simulink model "IEEE_BUS_68_AGC"  (R2025a)
settings: Solver=ode23tb  StartTime=0.0  StopTime=150  FixedStep=Ts  MaxStep=0.0001  RelTol=1e-3
PreLoadFcn:
  | PSSMODEL=1;
  | LPSS=0;
  | WAPSS=0;
  | WAPSS2=0;
  | Ts=50e-5;
InitFcn:
  | PSSMODEL=1;
  | LPSS=0;
  | WAPSS=0;
  | WAPSS2=0;
  | Ts=50e-5;
  | 
  | % Required data to 68 Bus benchmark
  | % clear
  | % clc
  | % Definition for the columns
  | % system base =100 MVA
  | 
  | %% Line data Format (line)
  | % All values are given on the same system base MVA
  | % 1: From bus
  | % 2: To bus
  | % 3: Resistance (pu)
  | % 4: Reactance  (pu)
  | % 5: Charge     (pu)
  | % 6: Transformer Tap Amplitute
  | % 7: base MVA
  | % 8: Nomonal Voltage (KV)
  | 
  | %1   2    3        4       5       6        7      8
  | line=[...
  | 1	54	0	     0.0181	  0	      1.025     100    13.8
  | 2	58	0	     0.025	  0	      1.070     100    13.8
  | 3	62	0	     0.02	  0	      1.070     100    13.8
  | 4	19	0.0007	 0.0142	  0	      1.070     100    13.8
  | 5	20	0.0009	 0.018	  0	      1.009     100    13.8
  | 6	22	0	     0.0143	  0	      1.025     100    13.8
  | 7	23	0.0005	 0.0272	  0	      0         100    13.8
  | 8	25	0.0006	 0.0232	  0	      1.025     100    13.8
  | 9	29	0.0008	 0.0156   0	      1.025     100    13.8
  | 10	31	0	     0.026	  0	      1.04      100    13.8
  | 11	32	0	     0.013	  0	      1.04      100    13.8
  | 12	36	0	     0.0075	  0	      1.04      100    13.8
  | 13	17	0	     0.0033	  0	      1.04      100    13.8
  | 14	41	0	     0.0015	  0	      1         100    13.8
  | 15	42	0	     0.0015	  0	      1         100    13.8
  | 16	18	0	     0.003	  0	      1         100    13.8
  | 17	36	0.0005	 0.0045	  0.32	  0         100    138
  | 17	43	0.0005	 0.0276	  0	      0         100    138
  | 18	42	0.004	 0.06	  2.25    0         100    138
  | 18	49	0.0076	 0.1141	  1.16    0	        100    138
  | 18	50	0.0012	 0.0288	  2.06	  0         100    138
  | 20	19	0.0007	 0.0138	  0       1.06	    100    138
  | 19	68	0.0016	 0.0195	  0.304	  0         100    138
  | 21	22	0.0008	 0.014	  0.2565  0	        100    138
  | 21	68	0.0008	 0.0135	  0.2548  0	        100    138
  | 22	23	0.0006	 0.0096	  0.1846  0	        100    138
  | 23	24	0.0022	 0.035	  0.361	  0         100    138
  | 24	68	0.0003	 0.0059	  0.068	  0         100    138
  | 25	26	0.0032	 0.0323	  0.531	  0         100    138
  | 25	54	0.007	 0.0086	  0.146	  0         100    138
  | 26	27	0.0014	 0.0147	  0.2396  0	        100    138
  | 26	28	0.0043	 0.0474	  0.7802  0	        100    138
  | 26	29	0.0057	 0.0625	  1.029	  0         100    138
  | 27	37	0.0013	 0.0173	  0.3216  0	        100    138
  | 27	53	0.032	 0.32	  0.41	  0         100    138
  | ... (+206 lines)
undefined symbols (not defined in the file or in its folder): D1, Delta
libraries: spsPMUPLLBasedPositiveSequenceLib x90, spsRMSLib x73, spsThreePhaseVIMeasurementLib x69, spsLoadFlowBusLib x69, spsThreePhasePISectionLineLib x64, spsThreePhaseParallelRLCLoadLib x35, spsGenericPowerSystemStabilizerLib x32, spsThreePhaseSeriesRLCLoadLib x21, spsThreePhaseTransformerTwoWindingsLib x21, spsSynchronousMachinepuStandardLib x20, spsExcitationSystemLib x16, spsMultiBandPowerSystemStabilizerLib x16
(part 4 of 8)

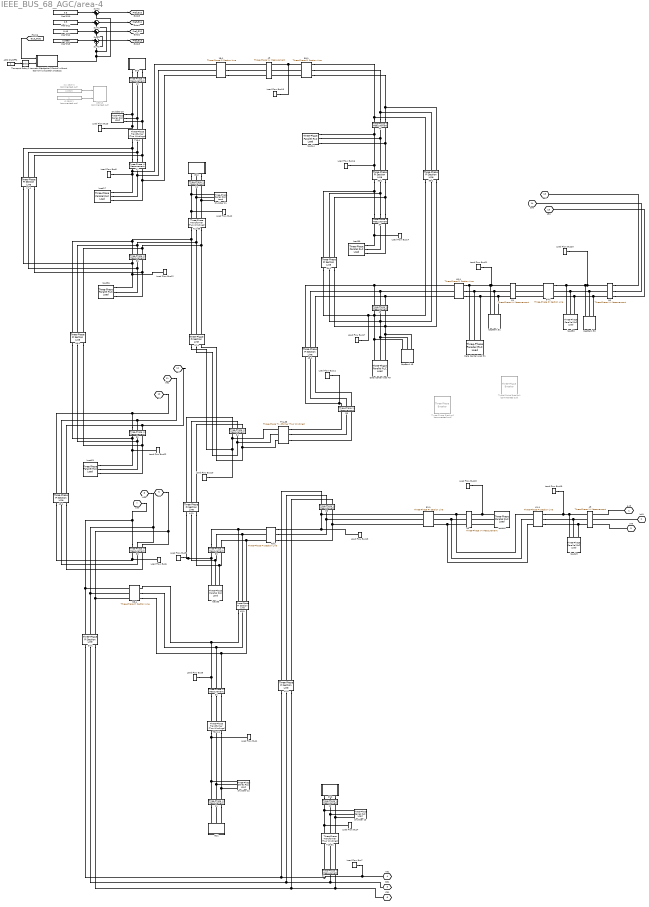
== system IEEE_BUS_68_AGC/area-4 ==
  10 : spsThreePhaseVIMeasurementLib/Three-Phase V-I Measurement  VoltageMeasurement=phase-to-phase  SetLabelV=on  LabelV=Vabc_10  Vpu=off  VpuLL=on  CurrentMeasurement=no  SetLabelI=off  LabelI=Iabc  Ipu=off  Pbase=100e6  Vbase=13.8e3  OutputType=Complex  PhasorSimulation=off  PSBequivalent=0
  11 : spsThreePhaseVIMeasurementLib/Three-Phase V-I Measurement  VoltageMeasurement=phase-to-phase  SetLabelV=on  LabelV=Vabc_11  Vpu=off  VpuLL=on  CurrentMeasurement=no  SetLabelI=off  LabelI=Iabc  Ipu=off  Pbase=100e6  Vbase=13.8e3  OutputType=Complex  PhasorSimulation=off  PSBequivalent=0
  12 : spsThreePhaseVIMeasurementLib/Three-Phase V-I Measurement  VoltageMeasurement=phase-to-phase  SetLabelV=on  LabelV=Vabc_12  Vpu=off  VpuLL=on  CurrentMeasurement=no  SetLabelI=off  LabelI=Iabc  Ipu=off  Pbase=100e6  Vbase=13.8e3  OutputType=Complex  PhasorSimulation=off  PSBequivalent=0
  13 : spsThreePhaseVIMeasurementLib/Three-Phase V-I Measurement  VoltageMeasurement=phase-to-phase  SetLabelV=on  LabelV=Vabc_13  Vpu=off  VpuLL=on  CurrentMeasurement=no  SetLabelI=off  LabelI=Iabc  Ipu=off  Pbase=100e6  Vbase=13.8e3  OutputType=Complex  PhasorSimulation=off  PSBequivalent=0
  17 : spsThreePhaseVIMeasurementLib/Three-Phase V-I Measurement  VoltageMeasurement=phase-to-phase  SetLabelV=on  LabelV=Vabc_17  Vpu=off  VpuLL=on  CurrentMeasurement=no  SetLabelI=off  LabelI=Iabc  Ipu=off  Pbase=100e6  Vbase=Bus(17,2)*1e3  OutputType=Complex  PhasorSimulation=off  PSBequivalent=0
  17-1 : spsThreePhasePISectionLineLib/Three-Phase PI Section Line  LConnTagsString=a|b|c  RConnTagsString=A|B|C  Length=1  Frequency=60  Resistances=[line(17,3) 3*line(17,3)]  Inductances=[line(17,4) 3*line(17,4)]  Capacitances=[line(17,5) line(17,5)/3]
  18-1 : spsThreePhasePISectionLineLib/Three-Phase PI Section Line  LConnTagsString=a|b|c  RConnTagsString=A|B|C  Length=1  Frequency=60  Resistances=[line(18,3) 3*line(18,3)]  Inductances=[line(18,4) 3*line(18,4)]  Capacitances=[line(28,5) line(28,5)/3]
  30 : spsThreePhaseVIMeasurementLib/Three-Phase V-I Measurement  VoltageMeasurement=phase-to-phase  SetLabelV=on  LabelV=Vabc_30  Vpu=off  VpuLL=on  CurrentMeasurement=no  SetLabelI=off  LabelI=Iabc  Ipu=off  Pbase=100e6  Vbase=Bus(30,2)*1e3  OutputType=Complex  PhasorSimulation=off  PSBequivalent=0
  31 : spsThreePhaseVIMeasurementLib/Three-Phase V-I Measurement  VoltageMeasurement=phase-to-phase  SetLabelV=on  LabelV=Vabc_31  Vpu=off  VpuLL=on  CurrentMeasurement=no  SetLabelI=off  LabelI=Iabc  Ipu=off  Pbase=100e6  Vbase=Bus(31,2)*1e3  OutputType=Complex  PhasorSimulation=off  PSBequivalent=0
  32 : spsThreePhaseVIMeasurementLib/Three-Phase V-I Measurement  VoltageMeasurement=phase-to-phase  SetLabelV=on  LabelV=Vabc_32  Vpu=off  VpuLL=on  CurrentMeasurement=no  SetLabelI=off  LabelI=Iabc  Ipu=off  Pbase=100e6  Vbase=Bus(32,2)*1e3  OutputType=Complex  PhasorSimulation=off  PSBequivalent=0
  33 : spsThreePhaseVIMeasurementLib/Three-Phase V-I Measurement  VoltageMeasurement=phase-to-phase  SetLabelV=on  LabelV=Vabc_33  Vpu=off  VpuLL=on  CurrentMeasurement=no  SetLabelI=off  LabelI=Iabc  Ipu=off  Pbase=100e6  Vbase=Bus(33,2)*1e3  OutputType=Complex  PhasorSimulation=off  PSBequivalent=0
  34 : spsThreePhaseVIMeasurementLib/Three-Phase V-I Measurement  VoltageMeasurement=phase-to-phase  SetLabelV=on  LabelV=Vabc_34  Vpu=off  VpuLL=on  CurrentMeasurement=no  SetLabelI=off  LabelI=Iabc  Ipu=off  Pbase=100e6  Vbase=Bus(34,2)*1e3  OutputType=Complex  PhasorSimulation=off  PSBequivalent=0
  35 : spsThreePhaseVIMeasurementLib/Three-Phase V-I Measurement  VoltageMeasurement=phase-to-phase  SetLabelV=on  LabelV=Vabc_35  Vpu=off  VpuLL=on  CurrentMeasurement=no  SetLabelI=off  LabelI=Iabc  Ipu=off  Pbase=100e6  Vbase=Bus(35,2)*1e3  OutputType=Complex  PhasorSimulation=off  PSBequivalent=0
  36 : spsThreePhaseVIMeasurementLib/Three-Phase V-I Measurement  VoltageMeasurement=phase-to-phase  SetLabelV=on  LabelV=Vabc_36  Vpu=off  VpuLL=on  CurrentMeasurement=no  SetLabelI=off  LabelI=Iabc  Ipu=off  Pbase=100e6  Vbase=Bus(36,2)*1e3  OutputType=Complex  PhasorSimulation=off  PSBequivalent=0
  37-1 : spsThreePhasePISectionLineLib/Three-Phase PI Section Line  LConnTagsString=a|b|c  RConnTagsString=A|B|C  Length=1  Frequency=60  Resistances=[line(37,3) 3*line(37,3)]  Inductances=[line(37,4) 3*line(37,4)]  Capacitances=[line(37,5) line(37,5)/3]
  38 : spsThreePhaseVIMeasurementLib/Three-Phase V-I Measurement  VoltageMeasurement=phase-to-phase  SetLabelV=on  LabelV=Vabc_38  Vpu=off  VpuLL=on  CurrentMeasurement=no  SetLabelI=off  LabelI=Iabc  Ipu=off  Pbase=100e6  Vbase=Bus(38,2)*1e3  OutputType=Complex  PhasorSimulation=off  PSBequivalent=0
  38-1 : spsThreePhasePISectionLineLib/Three-Phase PI Section Line  LConnTagsString=a|b|c  RConnTagsString=A|B|C  Length=1  Frequency=60  Resistances=[line(38,3) 3*line(38,3)]  Inductances=[line(38,4) 3*line(38,4)]  Capacitances=[line(38,5) line(38,5)/3]
  39 : spsThreePhaseVIMeasurementLib/Three-Phase V-I Measurement  VoltageMeasurement=phase-to-phase  SetLabelV=on  LabelV=Vabc_39  Vpu=off  VpuLL=on  CurrentMeasurement=no  SetLabelI=off  LabelI=Iabc  Ipu=off  Pbase=100e6  Vbase=Bus(39,2)*1e3  OutputType=Complex  PhasorSimulation=off  PSBequivalent=0
  40-1 : spsThreePhasePISectionLineLib/Three-Phase PI Section Line  LConnTagsString=a|b|c  RConnTagsString=A|B|C  Length=1  Frequency=60  Resistances=[line(40,3) 3*line(40,3)]  Inductances=[line(40,4) 3*line(40,4)]  Capacitances=[line(40,5) line(40,5)/3]
  41-1 : spsThreePhasePISectionLineLib/Three-Phase PI Section Line  LConnTagsString=a|b|c  RConnTagsString=A|B|C  Length=1  Frequency=60  Resistances=[line(45,3) 3*line(45,3)]  Inductances=[line(45,4) 3*line(45,4)]  Capacitances=[line(45,5) line(45,5)/3]
  43 : spsThreePhaseVIMeasurementLib/Three-Phase V-I Measurement  VoltageMeasurement=phase-to-phase  SetLabelV=on  LabelV=Vabc_43  Vpu=off  VpuLL=on  CurrentMeasurement=no  SetLabelI=off  LabelI=Iabc  Ipu=off  Pbase=100e6  Vbase=Bus(43,2)*1e3  OutputType=Complex  PhasorSimulation=off  PSBequivalent=0
  43-1 : spsThreePhasePISectionLineLib/Three-Phase PI Section Line  LConnTagsString=a|b|c  RConnTagsString=A|B|C  Length=1  Frequency=60  Resistances=[line(43,3) 3*line(43,3)]  Inductances=[line(43,4) 3*line(43,4)]  Capacitances=[line(43,5) line(43,5)/3]
  44 : spsThreePhaseVIMeasurementLib/Three-Phase V-I Measurement  VoltageMeasurement=phase-to-phase  SetLabelV=on  LabelV=Vabc_44  Vpu=off  VpuLL=on  CurrentMeasurement=no  SetLabelI=off  LabelI=Iabc  Ipu=off  Pbase=100e6  Vbase=Bus(44,2)*1e3  OutputType=Complex  PhasorSimulation=off  PSBequivalent=0
  44-1 : spsThreePhasePISectionLineLib/Three-Phase PI Section Line  LConnTagsString=a|b|c  RConnTagsString=A|B|C  Length=1  Frequency=60  Resistances=[line(44,3) 3*line(44,3)]  Inductances=[line(44,4) 3*line(44,4)]  Capacitances=[line(44,5) line(44,5)/3]
  45 : spsThreePhaseVIMeasurementLib/Three-Phase V-I Measurement  VoltageMeasurement=phase-to-phase  SetLabelV=on  LabelV=Vabc_45  Vpu=off  VpuLL=on  CurrentMeasurement=no  SetLabelI=off  LabelI=Iabc  Ipu=off  Pbase=100e6  Vbase=Bus(45,2)*1e3  OutputType=Complex  PhasorSimulation=off  PSBequivalent=0
  45-1 : spsThreePhasePISectionLineLib/Three-Phase PI Section Line  LConnTagsString=a|b|c  RConnTagsString=A|B|C  Length=1  Frequency=60  Resistances=[line(45,3) 3*line(45,3)]  Inductances=[line(45,4) 3*line(45,4)]  Capacitances=[line(45,5) line(45,5)/3]
  46 : spsThreePhaseVIMeasurementLib/Three-Phase V-I Measurement  VoltageMeasurement=phase-to-phase  SetLabelV=on  LabelV=Vabc_46  Vpu=off  VpuLL=on  CurrentMeasurement=no  SetLabelI=off  LabelI=Iabc  Ipu=off  Pbase=100e6  Vbase=Bus(46,2)*1e3  OutputType=Complex  PhasorSimulation=off  PSBequivalent=0
  47-1 : spsThreePhasePISectionLineLib/Three-Phase PI Section Line  LConnTagsString=a|b|c  RConnTagsString=A|B|C  Length=1  Frequency=60  Resistances=[line(47,3) 3*line(47,3)]  Inductances=[line(47,4) 3*line(47,4)]  Capacitances=[line(47,5) line(47,5)/3]
  48-1 : spsThreePhasePISectionLineLib/Three-Phase PI Section Line  LConnTagsString=a|b|c  RConnTagsString=A|B|C  Length=1  Frequency=60  Resistances=[line(48,3) 3*line(48,3)]  Inductances=[line(48,4) 3*line(48,4)]  Capacitances=[line(48,5) line(48,5)/3]
  49 : spsThreePhaseVIMeasurementLib/Three-Phase V-I Measurement  VoltageMeasurement=phase-to-phase  SetLabelV=on  LabelV=Vabc_49  Vpu=off  VpuLL=on  CurrentMeasurement=no  SetLabelI=off  LabelI=Iabc  Ipu=off  Pbase=100e6  Vbase=Bus(49,2)*1e3  OutputType=Complex  PhasorSimulation=off  PSBequivalent=0
  49-1 : spsThreePhasePISectionLineLib/Three-Phase PI Section Line  LConnTagsString=a|b|c  RConnTagsString=A|B|C  Length=1  Frequency=60  Resistances=[line(49,3) 3*line(49,3)]  Inductances=[line(49,4) 3*line(49,4)]  Capacitances=[line(49,5) line(49,5)/3]
  50 : spsThreePhaseVIMeasurementLib/Three-Phase V-I Measurement  VoltageMeasurement=phase-to-phase  SetLabelV=on  LabelV=Vabc_50  Vpu=off  VpuLL=on  CurrentMeasurement=no  SetLabelI=off  LabelI=Iabc  Ipu=off  Pbase=100e6  Vbase=Bus(50,2)*1e3  OutputType=Complex  PhasorSimulation=off  PSBequivalent=0
  51 : spsThreePhaseVIMeasurementLib/Three-Phase V-I Measurement  VoltageMeasurement=phase-to-phase  SetLabelV=on  LabelV=Vabc_51  Vpu=off  VpuLL=on  CurrentMeasurement=no  SetLabelI=off  LabelI=Iabc  Ipu=off  Pbase=100e6  Vbase=Bus(51,2)*1e3  OutputType=Complex  PhasorSimulation=off  PSBequivalent=0
  52-1 : spsThreePhasePISectionLineLib/Three-Phase PI Section Line  LConnTagsString=a|b|c  RConnTagsString=A|B|C  Length=1  Frequency=60  Resistances=[line(52,3) 3*line(52,3)]  Inductances=[line(52,4) 3*line(52,4)]  Capacitances=[line(52,5) line(52,5)/3]
  53-1 : spsThreePhasePISectionLineLib/Three-Phase PI Section Line  LConnTagsString=a|b|c  RConnTagsString=A|B|C  Length=1  Frequency=60  Resistances=[line(52,4) 3*line(52,4)]  Inductances=[line(53,4) 3*line(53,4)]  Capacitances=[line(28,5) line(28,5)/3]
  54-1 : spsThreePhasePISectionLineLib/Three-Phase PI Section Line  LConnTagsString=a|b|c  RConnTagsString=A|B|C  Length=1  Frequency=60  Resistances=[line(52,4) 3*line(52,4)]  Inductances=[line(54,4) 3*line(54,4)]  Capacitances=[line(28,5) line(28,5)/3]
  58-1 : spsThreePhasePISectionLineLib/Three-Phase PI Section Line  LConnTagsString=a|b|c  RConnTagsString=A|B|C  Length=1  Frequency=60  Resistances=[line(58,3) 3*line(58,3)]  Inductances=[line(58,4) 3*line(58,4)]  Capacitances=[line(28,5) line(28,5)/3]
  59-1 : spsThreePhasePISectionLineLib/Three-Phase PI Section Line  LConnTagsString=a|b|c  RConnTagsString=A|B|C  Length=1  Frequency=60  Resistances=[line(59,3) 3*line(59,3)]  Inductances=[line(59,4) 3*line(59,4)]  Capacitances=[line(28,5) line(28,5)/3]
  60-1 : spsThreePhasePISectionLineLib/Three-Phase PI Section Line  LConnTagsString=a|b|c  RConnTagsString=A|B|C  Length=1  Frequency=60  Resistances=[line(60,3) 3*line(60,3)]  Inductances=[line(60,4) 3*line(60,4)]  Capacitances=[line(60,5) line(60,5)/3]
  61 : spsThreePhaseVIMeasurementLib/Three-Phase V-I Measurement  VoltageMeasurement=phase-to-phase  SetLabelV=on  LabelV=Vabc_61  Vpu=off  VpuLL=on  CurrentMeasurement=no  SetLabelI=off  LabelI=Iabc  Ipu=off  Pbase=100e6  Vbase=Bus(61,2)*1e3  OutputType=Complex  PhasorSimulation=off  PSBequivalent=0
  61-1 : spsThreePhasePISectionLineLib/Three-Phase PI Section Line  LConnTagsString=a|b|c  RConnTagsString=A|B|C  Length=1  Frequency=60  Resistances=[line(61,3) 3*line(61,3)]  Inductances=[line(61,4) 3*line(61,4)]  Capacitances=[line(61,5) line(61,5)/3]
  64-1 : spsThreePhasePISectionLineLib/Three-Phase PI Section Line  LConnTagsString=a|b|c  RConnTagsString=A|B|C  Length=1  Frequency=60  Resistances=[line(64,3) 3*line(64,3)]  Inductances=[line(64,4) 3*line(64,4)]  Capacitances=[line(64,5) line(64,5)/3]
  AGC ON/OFF2 : Constant
  Automatic Generation Control without economic dispatch process2 : Subsystem
  CapBank 45 : spsThreePhaseSeriesRLCLoadLib/Three-Phase Series RLC Load  LConnTagsString=A|B|C  Configuration=Y (grounded)  NominalVoltage=138000  Vabc=[1e3 1e3 1e3]  Vabcp=[1e3 1e3 1e3]  NominalFrequency=60  UnbalancedPower=off  ActivePower=0  InductivePower=0  CapacitivePower=60000000  Pabc=[10e3 9e3 11e3]  QLabc=[100 90 110]  QCabc=[100 90 110]  Pabcp=[10e3 9e3 11e3]  QLabcp=[100 90 110]  QCabcp=[100 90 110]  Measurements=None  LoadType=constant Z
  CapBank 50 : spsThreePhaseSeriesRLCLoadLib/Three-Phase Series RLC Load  LConnTagsString=A|B|C  Configuration=Y (grounded)  NominalVoltage=138000  Vabc=[1e3 1e3 1e3]  Vabcp=[1e3 1e3 1e3]  NominalFrequency=60  UnbalancedPower=off  ActivePower=0  InductivePower=0  CapacitivePower=157000000  Pabc=[10e3 9e3 11e3]  QLabc=[100 90 110]  QCabc=[100 90 110]  Pabcp=[10e3 9e3 11e3]  QLabcp=[100 90 110]  QCabcp=[100 90 110]  Measurements=None  LoadType=constant Z
  CapBank 51 : spsThreePhaseSeriesRLCLoadLib/Three-Phase Series RLC Load  LConnTagsString=A|B|C  Configuration=Y (grounded)  NominalVoltage=138000  Vabc=[1e3 1e3 1e3]  Vabcp=[1e3 1e3 1e3]  NominalFrequency=60  UnbalancedPower=off  ActivePower=0  InductivePower=0  CapacitivePower=172000000  Pabc=[10e3 9e3 11e3]  QLabc=[100 90 110]  QCabc=[100 90 110]  Pabcp=[10e3 9e3 11e3]  QLabcp=[100 90 110]  QCabcp=[100 90 110]  Measurements=None  LoadType=constant Z
  Data Center Load 51 : spsThreePhaseParallelRLCLoadLib/Three-Phase Parallel RLC Load  LConnTagsString=A|B|C  Configuration=Y (grounded)  NominalVoltage=(138000)*0.99251  Vabc=[1e3 1e3 1e3]  Vabcp=[1e3 1e3 1e3]  NominalFrequency=60  UnbalancedPower=off  ActivePower=400000000  InductivePower=81200000  CapacitivePower=0  Pabc=[10e3 9e3 11e3]  QLabc=[100 90 110]  QCabc=[100 90 110]  Pabcp=[10e3 9e3 11e3]  QLabcp=[100 90 110]  QCabcp=[100 90 110]  Measurements=None  LoadType=constant PQ
  Data Center load 45 : spsThreePhaseParallelRLCLoadLib/Three-Phase Parallel RLC Load  LConnTagsString=A|B|C  Configuration=Y (grounded)  NominalVoltage=(138000)*0.982823  Vabc=[1e3 1e3 1e3]  Vabcp=[1e3 1e3 1e3]  NominalFrequency=60  UnbalancedPower=off  ActivePower=1000000000  InductivePower=203100000  CapacitivePower=0  Pabc=[10e3 9e3 11e3]  QLabc=[100 90 110]  QCabc=[100 90 110]  Pabcp=[10e3 9e3 11e3]  QLabcp=[100 90 110]  QCabcp=[100 90 110]  Measurements=None  LoadType=constant PQ
  G10 : Subsystem
  G11 : Subsystem
  G12 : Subsystem
  G13 : Subsystem
  Load Flow Bus1 : spsLoadFlowBusLib/Load Flow Bus  LConnTagsString=a  Phases=single  Connectors=on one side  ID=BUS_11  Vbase=13.8e3  Vref=1  Vangle=0  VLF=1  VLFb=1  VLFc=1  angleLF=-9.833  angleLFb=0  angleLFc=0
  Load Flow Bus10 : spsLoadFlowBusLib/Load Flow Bus  LConnTagsString=a  Phases=single  Connectors=on one side  ID=BUS_34  Vbase=138e3  Vref=1  Vangle=0  VLF=0.9874  VLFb=1  VLFc=1  angleLF=2.34  angleLFb=0  angleLFc=0
  Load Flow Bus11 : spsLoadFlowBusLib/Load Flow Bus  LConnTagsString=a  Phases=single  Connectors=on one side  ID=BUS_35  Vbase=138e3  Vref=1  Vangle=0  VLF=0.9889  VLFb=1  VLFc=1  angleLF=0.3546  angleLFb=0  angleLFc=0
  Load Flow Bus12 : spsLoadFlowBusLib/Load Flow Bus  LConnTagsString=a  Phases=single  Connectors=on one side  ID=BUS_36  Vbase=138e3  Vref=1  Vangle=0  VLF=0.9739  VLFb=1  VLFc=1  angleLF=1.118  angleLFb=0  angleLFc=0
  Load Flow Bus13 : spsLoadFlowBusLib/Load Flow Bus  LConnTagsString=a  Phases=single  Connectors=on one side  ID=BUS_38  Vbase=138e3  Vref=1  Vangle=0  VLF=1.017  VLFb=1  VLFc=1  angleLF=9.236  angleLFb=0  angleLFc=0
  Load Flow Bus14 : spsLoadFlowBusLib/Load Flow Bus  LConnTagsString=a  Phases=single  Connectors=on one side  ID=BUS_39  Vbase=138e3  Vref=1  Vangle=0  VLF=0.9805  VLFb=1  VLFc=1  angleLF=-5.956  angleLFb=0  angleLFc=0
  Load Flow Bus15 : spsLoadFlowBusLib/Load Flow Bus  LConnTagsString=a  Phases=single  Connectors=on one side  ID=BUS_43  Vbase=138e3  Vref=1  Vangle=0  VLF=0.9778  VLFb=1  VLFc=1  angleLF=-5.502  angleLFb=0  angleLFc=0
  Load Flow Bus16 : spsLoadFlowBusLib/Load Flow Bus  LConnTagsString=a  Phases=single  Connectors=on one side  ID=BUS_44  Vbase=138e3  Vref=1  Vangle=0  VLF=0.9779  VLFb=1  VLFc=1  angleLF=-5.529  angleLFb=0  angleLFc=0
  Load Flow Bus17 : spsLoadFlowBusLib/Load Flow Bus  LConnTagsString=a  Phases=single  Connectors=on one side  ID=BUS_45  Vbase=138e3  Vref=1  Vangle=0  VLF=0.9828  VLFb=1  VLFc=1  angleLF=-4.329  angleLFb=0  angleLFc=0
  Load Flow Bus18 : spsLoadFlowBusLib/Load Flow Bus  LConnTagsString=a  Phases=single  Connectors=on one side  ID=BUS_46  Vbase=138e3  Vref=1  Vangle=0  VLF=1.009  VLFb=1  VLFc=1  angleLF=8.853  angleLFb=0  angleLFc=0
  Load Flow Bus19 : spsLoadFlowBusLib/Load Flow Bus  LConnTagsString=a  Phases=single  Connectors=on one side  ID=BUS_49  Vbase=138e3  Vref=1  Vangle=0  VLF=1.003  VLFb=1  VLFc=1  angleLF=10.82  angleLFb=0  angleLFc=0
  Load Flow Bus2 : spsLoadFlowBusLib/Load Flow Bus  LConnTagsString=a  Phases=single  Connectors=on one side  ID=BUS_12  Vbase=13.8e3  Vref=1.0156  Vangle=0  VLF=1.016  VLFb=1  VLFc=1  angleLF=-22.82  angleLFb=0  angleLFc=0
  Load Flow Bus20 : spsLoadFlowBusLib/Load Flow Bus  LConnTagsString=a  Phases=single  Connectors=on one side  ID=BUS_50  Vbase=138e3  Vref=1  Vangle=0  VLF=1.001  VLFb=1  VLFc=1  angleLF=12.31  angleLFb=0  angleLFc=0
  Load Flow Bus21 : spsLoadFlowBusLib/Load Flow Bus  LConnTagsString=a  Phases=single  Connectors=on one side  ID=BUS_51  Vbase=138e3  Vref=1  Vangle=0  VLF=0.9925  VLFb=1  VLFc=1  angleLF=-0.6107  angleLFb=0  angleLFc=0
  Load Flow Bus22 : spsLoadFlowBusLib/Load Flow Bus  LConnTagsString=a  Phases=single  Connectors=on one side  ID=BUS_61  Vbase=138e3  Vref=1  Vangle=0  VLF=0.9818  VLFb=1  VLFc=1  angleLF=5.813  angleLFb=0  angleLFc=0
  Load Flow Bus3 : spsLoadFlowBusLib/Load Flow Bus  LConnTagsString=a  Phases=single  Connectors=on one side  ID=BUS_13  Vbase=13.8e3  Vref=1.011  Vangle=0  VLF=1.011  VLFb=1  VLFc=1  angleLF=-28.14  angleLFb=0  angleLFc=0
  Load Flow Bus4 : spsLoadFlowBusLib/Load Flow Bus  LConnTagsString=a  Phases=single  Connectors=on one side  ID=BUS_10  Vbase=13.8e3  Vref=1.01  Vangle=0  VLF=1.01  VLFb=1  VLFc=1  angleLF=-11.9  angleLFb=0  angleLFc=0
  Load Flow Bus5 : spsLoadFlowBusLib/Load Flow Bus  LConnTagsString=a  Phases=single  Connectors=on one side  ID=BUS_17  Vbase=138e3  Vref=1  Vangle=0  VLF=0.971  VLFb=1  VLFc=1  angleLF=-4.835  angleLFb=0  angleLFc=0
  Load Flow Bus6 : spsLoadFlowBusLib/Load Flow Bus  LConnTagsString=a  Phases=single  Connectors=on one side  ID=BUS_30  Vbase=138e3  Vref=1  Vangle=0  VLF=1.002  VLFb=1  VLFc=1  angleLF=8.559  angleLFb=0  angleLFc=0
  Load Flow Bus7 : spsLoadFlowBusLib/Load Flow Bus  LConnTagsString=a  Phases=single  Connectors=on one side  ID=BUS_31  Vbase=138e3  Vref=1  Vangle=0  VLF=1.012  VLFb=1  VLFc=1  angleLF=10.81  angleLFb=0  angleLFc=0
  Load Flow Bus8 : spsLoadFlowBusLib/Load Flow Bus  LConnTagsString=a  Phases=single  Connectors=on one side  ID=BUS_32  Vbase=138e3  Vref=1  Vangle=0  VLF=0.997  VLFb=1  VLFc=1  angleLF=12.7  angleLFb=0  angleLFc=0
  Load Flow Bus9 : spsLoadFlowBusLib/Load Flow Bus  LConnTagsString=a  Phases=single  Connectors=on one side  ID=BUS_33  Vbase=138e3  Vref=1  Vangle=0  VLF=0.9947  VLFb=1  VLFc=1  angleLF=8.424  angleLFb=0  angleLFc=0
  Pm REG13 : Constant  Commented=on  Value=0.8929
  Pref G10 : Constant  Value=0.5
  Pref G11 : Constant  Value=0.5
  Pref G12 : Constant  Value=0.45
  Pref G13 : Constant  Value=0.5985
  REG13 : spsSynchronousMachinepuStandardLib/Synchronous Machine pu Standard  Commented=on  PresetModel=No  MechanicalLoad=Mechanical power Pm  ShowDetailedParameters=on  RotorType=Round  Units=per unit standard parameters  MeasurementBus=off  NominalParameters="[ 721.4e6  13800  60 ]"  Reactances1="[mac_con(13,6:8)  mac_con(13,11:13)  mac_con(13,4)]"  Reactances2=[ 1.305, 0.296, 0.252, 0.474, 0.243, 0.18 ]  dAxisTimeConstants=Open-circuit  qAxisTimeConstants=Open-circuit  TimeConstants1=[]  TimeConstants2="[mac_con(13,9:10)  mac_con(13,14:15)]"  TimeConstants3=[]  TimeConstants4=[]  TimeConstants5=[ 1.01, 0.053, 0.1 ]  TimeConstants6=[]  TimeConstants7=[]  TimeConstants8=[]  StatorResistance=mac_con(13,5)  Mechanical=[ 1.0 0 4 ]  PolePairs=4  InitialConditions=[0 -110.907 0.613873 0.613873 0.613873 -37.2072 -157.207 82.7928 1.01596]  SetSaturation=off  Saturation=[0.6404,0.7127,0.8441,0.9214,0.9956,1.082,1.19,1.316,1.457;0.7,0.7698,0.8872,0.9466,0.9969,1.046,1.1,1.151,1.201]  LoadFlowParameters=[1 830000000 0 0 0]  TsPowergui=0  TsBlock=-1  IterativeModel=Trapezoidal non iterative  IterativeDiscreteModel=Trapezoidal non iterative  BusType=PQ  Pref=644.1e6  Qref=0  Qmin=-Inf  Qmax=Inf  PLF=0  QLF=0
  Snubber {10..13} (4 alike) : spsThreePhaseSeriesRLCLoadLib/Three-Phase Series RLC Load  LConnTagsString=A|B|C  Configuration=Y (grounded)  NominalVoltage=13.8e3  Vabc=[1e3 1e3 1e3]  Vabcp=[1e3 1e3 1e3]  NominalFrequency=60  UnbalancedPower=off  ActivePower=1000000  InductivePower=0  CapacitivePower=10000000  Pabc=[10e3 9e3 11e3]  QLabc=[100 90 110]  QCabc=[100 90 110]  Pabcp=[10e3 9e3 11e3]  QLabcp=[100 90 110]  QCabcp=[100 90 110]  Measurements=None  LoadType=constant Z
  Sum{1..2,4..5} (4 alike) : Sum  Inputs=|++
  T10-31 : spsThreePhaseTransformerTwoWindingsLib/Three-Phase Transformer (Two Windings)  Winding1Connection=Delta (D1)  Winding2Connection=Yg  CoreType=Three single-phase transformers  SetSaturation=off  Hysteresis=off  DataFile='hysteresis'  SetInitialFlux=off  Measurements=None  UNITS=pu  NominalPower=[ 100e6 , 60 ]  Winding1=[ 13.8e3 , 0.0002 , 0 ]  Winding2=[ 138e3 , 0.0002 , 0.026 ]  Rm=500  Lm=500  L0=0.5  Saturation=[ 0,0 ; 0.0024,1.2 ; 1.0,1.52 ]  InitialFluxes=[ 0.8 , -0.8 , 0.7 ]  BreakLoop=off  DiscreteSolver=Trapezoidal robust  DataType=off  TransfoNumber=1
  T12-36 : spsThreePhaseTransformerTwoWindingsLib/Three-Phase Transformer (Two Windings)  Winding1Connection=Delta (D1)  Winding2Connection=Yg  CoreType=Three single-phase transformers  SetSaturation=off  Hysteresis=off  DataFile='hysteresis'  SetInitialFlux=off  Measurements=None  UNITS=pu  NominalPower=[ 100e6 , 60 ]  Winding1=[ 13.8e3 , 0.002 , 0 ]  Winding2=[ 138e3 , 0.002 , 0.0075 ]  Rm=500  Lm=500  L0=0.5  Saturation=[ 0,0 ; 0.0024,1.2 ; 1.0,1.52 ]  InitialFluxes=[ 0.8 , -0.8 , 0.7 ]  BreakLoop=off  DiscreteSolver=Trapezoidal robust  DataType=off  TransfoNumber=1
  T13-1 : spsThreePhaseTransformerTwoWindingsLib/Three-Phase Transformer (Two Windings)  Winding1Connection=Delta (D1)  Winding2Connection=Yg  CoreType=Three single-phase transformers  SetSaturation=off  Hysteresis=off  DataFile='hysteresis'  SetInitialFlux=off  Measurements=None  UNITS=pu  NominalPower=[ 100e6 , 60 ]  Winding1=[ 13.8e3 , 0.0002 , 0 ]  Winding2=[ 138e3 , 0.0002, 0.0033 ]  Rm=500  Lm=500  L0=0.5  Saturation=[ 0,0 ; 0.0024,1.2 ; 1.0,1.52 ]  InitialFluxes=[ 0.8 , -0.8 , 0.7 ]  BreakLoop=off  DiscreteSolver=Trapezoidal robust  DataType=off  TransfoNumber=1
  T32-11 : spsThreePhaseTransformerTwoWindingsLib/Three-Phase Transformer (Two Windings)  Winding1Connection=Delta (D1)  Winding2Connection=Yg  CoreType=Three single-phase transformers  SetSaturation=off  Hysteresis=off  DataFile='hysteresis'  SetInitialFlux=off  Measurements=None  UNITS=pu  NominalPower=[ 100e6 , 60 ]  Winding1=[ 13.8e3 , 0.00020 , 0 ]  Winding2=[ 138e3 , 0.0002 , 0.013 ]  Rm=500  Lm=500  L0=0.5  Saturation=[ 0,0 ; 0.0024,1.2 ; 1.0,1.52 ]  InitialFluxes=[ 0.8 , -0.8 , 0.7 ]  BreakLoop=off  DiscreteSolver=Trapezoidal robust  DataType=off  TransfoNumber=1
  T34-35 : spsThreePhaseTransformerTwoWindingsLib/Three-Phase Transformer (Two Windings)  Winding1Connection=Y  Winding2Connection=Y  CoreType=Three single-phase transformers  SetSaturation=off  Hysteresis=off  DataFile='hysteresis'  SetInitialFlux=off  Measurements=None  UNITS=pu  NominalPower=[ 100e6 , 60 ]  Winding1=[ 138e3 , 0.00005 , 0 ]  Winding2=[ 138e3 , 0.00005 , 0.0074 ]  Rm=500  Lm=500  L0=0.5  Saturation=[ 0,0 ; 0.0024,1.2 ; 1.0,1.52 ]  InitialFluxes=[ 0.8 , -0.8 , 0.7 ]  BreakLoop=off  DiscreteSolver=Trapezoidal robust  DataType=off  TransfoNumber=1
  Three-Phase Breaker1 : spsThreePhaseBreakerLib/Three-Phase Breaker  Commented=on  InitialState=closed  SwitchA=on  SwitchB=on  SwitchC=on  SwitchTimes=11.975  External=off  BreakerResistance=0.01  SnubberResistance=1e6  SnubberCapacitance=inf  Measurements=None
  Three-Phase Breaker2 : spsThreePhaseBreakerLib/Three-Phase Breaker  Commented=on  InitialState=closed  SwitchA=on  SwitchB=on  SwitchC=on  SwitchTimes=5  External=off  BreakerResistance=0.01  SnubberResistance=1e6  SnubberCapacitance=inf  Measurements=None
  Transport Delay2 : TransportDelay  DelayTime=20
  Vf REG13 : Constant  Commented=on
  load17 : spsThreePhaseParallelRLCLoadLib/Three-Phase Parallel RLC Load  LConnTagsString=A|B|C  Configuration=Y (grounded)  NominalVoltage=(138000)*0.970987  Vabc=[1e3 1e3 1e3]  Vabcp=[1e3 1e3 1e3]  NominalFrequency=60  UnbalancedPower=off  ActivePower=5643000000  InductivePower=300000000  CapacitivePower=0  Pabc=[10e3 9e3 11e3]  QLabc=[100 90 110]  QCabc=[100 90 110]  Pabcp=[10e3 9e3 11e3]  QLabcp=[100 90 110]  QCabcp=[100 90 110]  Measurements=None  LoadType=constant PQ
  load33 : spsThreePhaseParallelRLCLoadLib/Three-Phase Parallel RLC Load  LConnTagsString=A|B|C  Configuration=Y (grounded)  NominalVoltage=(138000)*0.994743  Vabc=[1e3 1e3 1e3]  Vabcp=[1e3 1e3 1e3]  NominalFrequency=60  UnbalancedPower=off  ActivePower=112000000  InductivePower=0  CapacitivePower=0  Pabc=[10e3 9e3 11e3]  QLabc=[100 90 110]  QCabc=[100 90 110]  Pabcp=[10e3 9e3 11e3]  QLabcp=[100 90 110]  QCabcp=[100 90 110]  Measurements=None  LoadType=constant PQ
  load36 : spsThreePhaseParallelRLCLoadLib/Three-Phase Parallel RLC Load  LConnTagsString=A|B|C  Configuration=Y (grounded)  NominalVoltage=(138000)*0.973922  Vabc=[1e3 1e3 1e3]  Vabcp=[1e3 1e3 1e3]  NominalFrequency=60  UnbalancedPower=off  ActivePower=102000000  InductivePower=0  CapacitivePower=19600000  Pabc=[10e3 9e3 11e3]  QLabc=[100 90 110]  QCabc=[100 90 110]  Pabcp=[10e3 9e3 11e3]  QLabcp=[100 90 110]  QCabcp=[100 90 110]  Measurements=None  LoadType=constant PQ
  load39 : spsThreePhaseParallelRLCLoadLib/Three-Phase Parallel RLC Load  LConnTagsString=A|B|C  Configuration=Y (grounded)  NominalVoltage=(138000)*0.980486  Vabc=[1e3 1e3 1e3]  Vabcp=[1e3 1e3 1e3]  NominalFrequency=60  UnbalancedPower=off  ActivePower=50000000  InductivePower=2600000  CapacitivePower=0  Pabc=[10e3 9e3 11e3]  QLabc=[100 90 110]  QCabc=[100 90 110]  Pabcp=[10e3 9e3 11e3]  QLabcp=[100 90 110]  QCabcp=[100 90 110]  Measurements=None  LoadType=constant PQ
  load44 : spsThreePhaseParallelRLCLoadLib/Three-Phase Parallel RLC Load  LConnTagsString=A|B|C  Configuration=Y (grounded)  NominalVoltage=(138000)*0.977937  Vabc=[1e3 1e3 1e3]  Vabcp=[1e3 1e3 1e3]  NominalFrequency=60  UnbalancedPower=off  ActivePower=50000000  InductivePower=2600000  CapacitivePower=0  Pabc=[10e3 9e3 11e3]  QLabc=[100 90 110]  QCabc=[100 90 110]  Pabcp=[10e3 9e3 11e3]  QLabcp=[100 90 110]  QCabcp=[100 90 110]  Measurements=None  LoadType=constant PQ
  load46 : spsThreePhaseParallelRLCLoadLib/Three-Phase Parallel RLC Load  LConnTagsString=A|B|C  Configuration=Y (grounded)  NominalVoltage=(138000)*1.00927  Vabc=[1e3 1e3 1e3]  Vabcp=[1e3 1e3 1e3]  NominalFrequency=60  UnbalancedPower=off  ActivePower=151000000  InductivePower=28000000  CapacitivePower=0  Pabc=[10e3 9e3 11e3]  QLabc=[100 90 110]  QCabc=[100 90 110]  Pabcp=[10e3 9e3 11e3]  QLabcp=[100 90 110]  QCabcp=[100 90 110]  Measurements=None  LoadType=constant PQ
  load49 : spsThreePhaseParallelRLCLoadLib/Three-Phase Parallel RLC Load  LConnTagsString=A|B|C  Configuration=Y (grounded)  NominalVoltage=(138000)*1.00283  Vabc=[1e3 1e3 1e3]  Vabcp=[1e3 1e3 1e3]  NominalFrequency=60  UnbalancedPower=off  ActivePower=164000000  InductivePower=29000000  CapacitivePower=0  Pabc=[10e3 9e3 11e3]  QLabc=[100 90 110]  QCabc=[100 90 110]  Pabcp=[10e3 9e3 11e3]  QLabcp=[100 90 110]  QCabcp=[100 90 110]  Measurements=None  LoadType=constant PQ
  load50 : spsThreePhaseParallelRLCLoadLib/Three-Phase Parallel RLC Load  LConnTagsString=A|B|C  Configuration=Y (grounded)  NominalVoltage=(138000)*1.00129  Vabc=[1e3 1e3 1e3]  Vabcp=[1e3 1e3 1e3]  NominalFrequency=60  UnbalancedPower=off  ActivePower=37000000  InductivePower=7500000  CapacitivePower=0  Pabc=[10e3 9e3 11e3]  QLabc=[100 90 110]  QCabc=[100 90 110]  Pabcp=[10e3 9e3 11e3]  QLabcp=[100 90 110]  QCabcp=[100 90 110]  Measurements=None  LoadType=constant PQ
  load61 : spsThreePhaseParallelRLCLoadLib/Three-Phase Parallel RLC Load  LConnTagsString=A|B|C  Configuration=Y (grounded)  NominalVoltage=(138000)*0.981797  Vabc=[1e3 1e3 1e3]  Vabcp=[1e3 1e3 1e3]  NominalFrequency=60  UnbalancedPower=off  ActivePower=104000000  InductivePower=125000000  CapacitivePower=0  Pabc=[10e3 9e3 11e3]  QLabc=[100 90 110]  QCabc=[100 90 110]  Pabcp=[10e3 9e3 11e3]  QLabcp=[100 90 110]  QCabcp=[100 90 110]  Measurements=None  LoadType=constant PQ
  a49 : PMIOPort  Tag=PMCPort  Side=Right
  b49 : PMIOPort  Tag=PMCPort  Port=2  Side=Right
  c49 : PMIOPort  Tag=PMCPort  Port=3  Side=Right
  A31 : PMIOPort  Tag=PMCPort  Port=4  Side=Right
  B31 : PMIOPort  Tag=PMCPort  Port=5  Side=Right
  C31 : PMIOPort  Tag=PMCPort  Port=6  Side=Right
  a30 : PMIOPort  Tag=PMCPort  Port=7  Side=Right
  b30 : PMIOPort  Tag=PMCPort  Port=8  Side=Right
  c30 : PMIOPort  Tag=PMCPort  Port=9  Side=Right
  a61 : PMIOPort  Tag=PMCPort  Port=10  Side=Right
  b61 : PMIOPort  Tag=PMCPort  Port=11  Side=Right
  c61 : PMIOPort  Tag=PMCPort  Port=12  Side=Right
  a50 : PMIOPort  Tag=PMCPort  Port=13  Side=Right
  b50 : PMIOPort  Tag=PMCPort  Port=14  Side=Right
  c50 : PMIOPort  Tag=PMCPort  Port=15  Side=Right
  tag scope: Pref_G10=global, Pref_G11=global, Pref_G12=global, Pref_G13=global
  wires:
  Automatic Generation Control without economic dispatch process2/1(Delta_P) -> Sum2/2, Sum1/2, Sum4/2, Sum5/2
  Transport Delay2/1 -> Automatic Generation Control without economic dispatch process2/2(AGC Status)
  Pref G13/1 -> Sum5/1
  Pref G12/1 -> Sum4/1
  AGC ON/OFF2/1 -> Transport Delay2/1
  [G13_Goto] -> Automatic Generation Control without economic dispatch process2/1(dw)
  Pref G10/1 -> Sum2/1
  Pref G11/1 -> Sum1/1
  Sum2/1 -> [Pref_G10]
  Sum1/1 -> [Pref_G11]
  Sum4/1 -> [Pref_G12]
  Sum5/1 -> [Pref_G13]
  Pm REG13/1 -> REG13/1
  Vf REG13/1 -> REG13/2
  connections:
  G13/LConn1 -- 13/RConn1
  T13-1/LConn1 -- Load Flow Bus3/LConn1 -- 13/LConn1 -- Snubber 10/LConn1
  17/RConn2 -- T13-1/RConn2 -- 17-1/LConn2
  G13/LConn3 -- 13/RConn3
  G13/LConn2 -- 13/RConn2
  T13-1/RConn3 -- 17/RConn3 -- 17-1/LConn3
  17/RConn1 -- T13-1/RConn1 -- 17-1/LConn1
  load17/LConn1 -- Load Flow Bus5/LConn1 -- 17/LConn1 -- 18-1/RConn1
  load17/LConn2 -- 17/LConn2 -- 18-1/RConn2
  load17/LConn3 -- 18-1/RConn3 -- 17/LConn3
  49-1/LConn1 -- 36/RConn1 -- 47-1/LConn1 -- T12-36/RConn1
  T12-36/RConn2 -- 49-1/LConn2 -- 36/RConn2 -- 47-1/LConn2
  T12-36/RConn3 -- 49-1/LConn3 -- 36/RConn3 -- 47-1/LConn3
  G12/LConn1 -- 12/RConn1
  G12/LConn2 -- 12/RConn2
  G12/LConn3 -- 12/RConn3
  T12-36/LConn1 -- Load Flow Bus2/LConn1 -- Snubber 11/LConn1 -- 12/LConn1
  T12-36/LConn2 -- 12/LConn2 -- Snubber 11/LConn2
  T12-36/LConn3 -- Snubber 11/LConn3 -- 12/LConn3
  load36/LConn1 -- Load Flow Bus12/LConn1 -- 17-1/RConn1 -- 36/LConn1
  load36/LConn2 -- 17-1/RConn2 -- 36/LConn2
  load36/LConn3 -- 17-1/RConn3 -- 36/LConn3
  61/RConn1 -- a61/RConn1 -- 40-1/LConn1
  b61/RConn1 -- 61/RConn2 -- 40-1/LConn2
  c61/RConn1 -- 61/RConn3 -- 40-1/LConn3
  load61/LConn1 -- Load Flow Bus22/LConn1 -- 61/LConn1 -- 49-1/RConn1
  load61/LConn2 -- 61/LConn2 -- 49-1/RConn2
  load61/LConn3 -- 61/LConn3 -- 49-1/RConn3
  30/RConn1 -- a30/RConn1 -- 38-1/LConn1 -- 37-1/LConn1
  37-1/LConn2 -- 30/RConn2 -- b30/RConn1 -- 38-1/LConn2
  37-1/LConn3 -- 30/RConn3 -- c30/RConn1 -- 38-1/LConn3
  47-1/RConn1 -- 34/LConn1 -- T34-35/LConn1 -- Load Flow Bus10/LConn1
  47-1/RConn2 -- T34-35/LConn2 -- 34/LConn2
  47-1/RConn3 -- T34-35/LConn3 -- 34/LConn3
  33/RConn1 -- 45-1/LConn1 -- 43-1/LConn1
  45-1/LConn2 -- 33/RConn2 -- 43-1/LConn2
  45-1/LConn3 -- 33/RConn3 -- 43-1/LConn3
  44-1/RConn1 -- Load Flow Bus9/LConn1 -- 33/LConn1 -- load33/LConn1
  load33/LConn2 -- 44-1/RConn2 -- 33/LConn2
  33/LConn3 -- 44-1/RConn3 -- load33/LConn3
  38-1/RConn1 -- Load Flow Bus8/LConn1 -- 32/LConn1 -- 43-1/RConn1
  32/LConn2 -- 38-1/RConn2 -- 43-1/RConn2
  32/LConn3 -- 38-1/RConn3 -- 43-1/RConn3
  40-1/RConn1 -- Load Flow Bus6/LConn1 -- 30/LConn1
  40-1/RConn2 -- 30/LConn2
  40-1/RConn3 -- 30/LConn3
  11/RConn1 -- G11/LConn1
  45-1/RConn1 -- Load Flow Bus13/LConn1 -- 38/LConn1 -- 52-1/RConn1
  38/LConn2 -- 45-1/RConn2 -- 52-1/RConn2
  38/LConn3 -- 45-1/RConn3 -- 52-1/RConn3
  G10/LConn1 -- 10/RConn1
  G10/LConn2 -- 10/RConn2
  G10/LConn3 -- 10/RConn3
  T10-31/LConn1 -- Load Flow Bus4/LConn1 -- Snubber 13/LConn1 -- 10/LConn1
  T10-31/LConn2 -- 10/LConn2 -- Snubber 13/LConn2
  T10-31/LConn3 -- Snubber 13/LConn3 -- 10/LConn3
  31/RConn1 -- T10-31/RConn1
  31/RConn2 -- T10-31/RConn2
  31/RConn3 -- T10-31/RConn3
  41-1/LConn1 -- 38/RConn1
  41-1/LConn2 -- 38/RConn2
  41-1/LConn3 -- 38/RConn3
  43/RConn1 -- 18-1/LConn1
  18-1/LConn2 -- 43/RConn2
  18-1/LConn3 -- 43/RConn3
  58-1/RConn1 -- Load Flow Bus15/LConn1 -- 43/LConn1
  58-1/RConn2 -- 43/LConn2
  58-1/RConn3 -- 43/LConn3
  44/RConn1 -- 58-1/LConn1 -- 59-1/LConn1
  44/RConn2 -- 58-1/LConn2 -- 59-1/LConn2
  44/RConn3 -- 58-1/LConn3 -- 59-1/LConn3
  53-1/RConn1 -- load44/LConn1 -- 44/LConn1 -- Load Flow Bus16/LConn1
  53-1/RConn2 -- load44/LConn2 -- 44/LConn2
  53-1/RConn3 -- load44/LConn3 -- 44/LConn3
  39/RConn1 -- 53-1/LConn1 -- 54-1/LConn1
  39/RConn2 -- 53-1/LConn2 -- 54-1/LConn2
  39/RConn3 -- 53-1/LConn3 -- 54-1/LConn3
  Load Flow Bus14/LConn1 -- load39/LConn1 -- 39/LConn1
  60-1/LConn1 -- 45/RConn1 -- 48-1/LConn1
  60-1/LConn2 -- 48-1/LConn2 -- 45/RConn2
  60-1/LConn3 -- 48-1/LConn3 -- 45/RConn3
  Load Flow Bus17/LConn1 -- Data Center load 45/LConn1 -- CapBank 45/LConn1 -- 59-1/RConn1 -- 45/LConn1 -- 54-1/RConn1
  35/LConn1 -- Load Flow Bus11/LConn1 -- 48-1/RConn1
  35/LConn2 -- 48-1/RConn2
  35/LConn3 -- 48-1/RConn3
  A31/RConn1 -- Load Flow Bus7/LConn1 -- 31/LConn1 -- 41-1/RConn1 -- 37-1/RConn1
  B31/RConn1 -- 31/LConn2 -- 41-1/RConn2 -- 37-1/RConn2
  C31/RConn1 -- 31/LConn3 -- 41-1/RConn3 -- 37-1/RConn3
  60-1/RConn1 -- Data Center Load 51/LConn1 -- CapBank 51/LConn1 -- 51/LConn1 -- Load Flow Bus21/LConn1
  60-1/RConn2 -- Data Center Load 51/LConn2 -- 51/LConn2 -- CapBank 51/LConn2
  60-1/RConn3 -- Data Center Load 51/LConn3 -- CapBank 51/LConn3 -- 51/LConn3
  64-1/LConn1 -- 51/RConn1
  64-1/LConn2 -- 51/RConn2
  64-1/LConn3 -- 51/RConn3
  64-1/RConn1 -- CapBank 50/LConn1 -- 50/LConn1 -- Load Flow Bus20/LConn1 -- load50/LConn1
  50/LConn2 -- load50/LConn2 -- 64-1/RConn2 -- CapBank 50/LConn2
  50/LConn3 -- load50/LConn3 -- 64-1/RConn3 -- CapBank 50/LConn3
  50/RConn1 -- a50/RConn1
  50/RConn2 -- b50/RConn1
  50/RConn3 -- c50/RConn1
  61-1/RConn1 -- Load Flow Bus19/LConn1 -- load49/LConn1 -- 49/LConn1
  61-1/RConn2 -- load49/LConn2 -- 49/LConn2
  61-1/RConn3 -- load49/LConn3 -- 49/LConn3
  c49/RConn1 -- 49/RConn3
  b49/RConn1 -- 49/RConn2
  a49/RConn1 -- 49/RConn1
  32/RConn1 -- T32-11/RConn1
  32/RConn2 -- T32-11/RConn2
  32/RConn3 -- T32-11/RConn3
  T32-11/LConn1 -- Snubber 12/LConn1 -- 11/LConn1 -- Load Flow Bus1/LConn1
  T32-11/LConn2 -- 11/LConn2 -- Snubber 12/LConn2
  T32-11/LConn3 -- Snubber 12/LConn3 -- 11/LConn3
  11/RConn2 -- G11/LConn2
  11/RConn3 -- G11/LConn3
  T13-1/LConn2 -- 13/LConn2 -- Snubber 10/LConn2
  T13-1/LConn3 -- 13/LConn3 -- Snubber 10/LConn3
  T34-35/RConn1 -- 35/RConn1
  T34-35/RConn2 -- 35/RConn2
  T34-35/RConn3 -- 35/RConn3
  44-1/LConn3 -- 34/RConn3
  44-1/LConn2 -- 34/RConn2
  44-1/LConn1 -- 34/RConn1
  46/RConn1 -- 52-1/LConn1 -- 61-1/LConn1
  46/RConn2 -- 52-1/LConn2 -- 61-1/LConn2
  52-1/LConn3 -- 46/RConn3 -- 61-1/LConn3
  load46/LConn1 -- Load Flow Bus18/LConn1 -- 46/LConn1
  load46/LConn2 -- 46/LConn2
  load46/LConn3 -- 46/LConn3
  54-1/RConn2 -- Data Center load 45/LConn2 -- CapBank 45/LConn2 -- 45/LConn2 -- 59-1/RConn2
  54-1/RConn3 -- Data Center load 45/LConn3 -- CapBank 45/LConn3 -- 59-1/RConn3 -- 45/LConn3
  load39/LConn2 -- 39/LConn2
  load39/LConn3 -- 39/LConn3
